simulink model "exp1_2"  (R2018b)
settings: Solver=VariableStepAuto  StartTime=0.0  StopTime=10.0  RelTol=1e-3
settings Model: Creator=lenovo  LastModifiedBy=lenovo

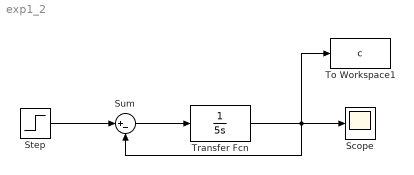
== system exp1_2 ==
  Scope : Scope
  Step : Step  SampleTime=0
  Sum : Sum  Inputs=|+-
  To Workspace1 : ToWorkspace  VariableName=c  SaveFormat=Structure With Time  SampleTime=-1
  Transfer Fcn : TransferFcn  Denominator=[5 0]
  wires:
  Transfer Fcn/1 -> To Workspace1/1, Sum/2, Scope/1
  Step/1 -> Sum/1
  Sum/1 -> Transfer Fcn/1
